simulink model "LC_DAB"  (R2025a)
settings: Solver=VariableStepAuto  StartTime=0.0  StopTime=1  RelTol=1e-3
libraries: spsVoltageMeasurementLib x5, spsCurrentMeasurementLib x4, spsIGBTDiodeLib x4, spsMosfetLib x4, spsSeriesRLCBranchLib x4, spsMeanLib x2, spsDCVoltageSourceLib x1, spsLinearTransformerLib x1, sps_lib x1
settings Model: Creator=hp  LastModifiedBy=photortist

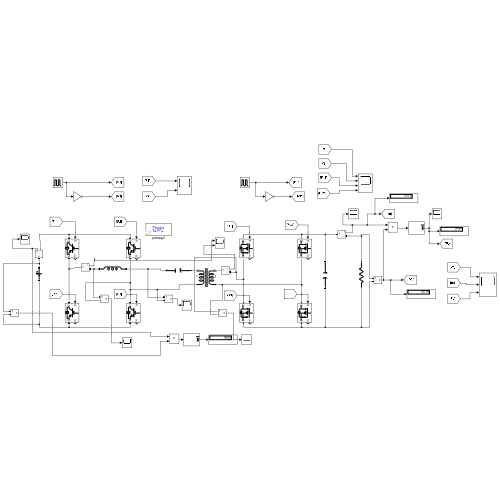
[thumbnail: Simulink's stored preview of the top-level diagram]
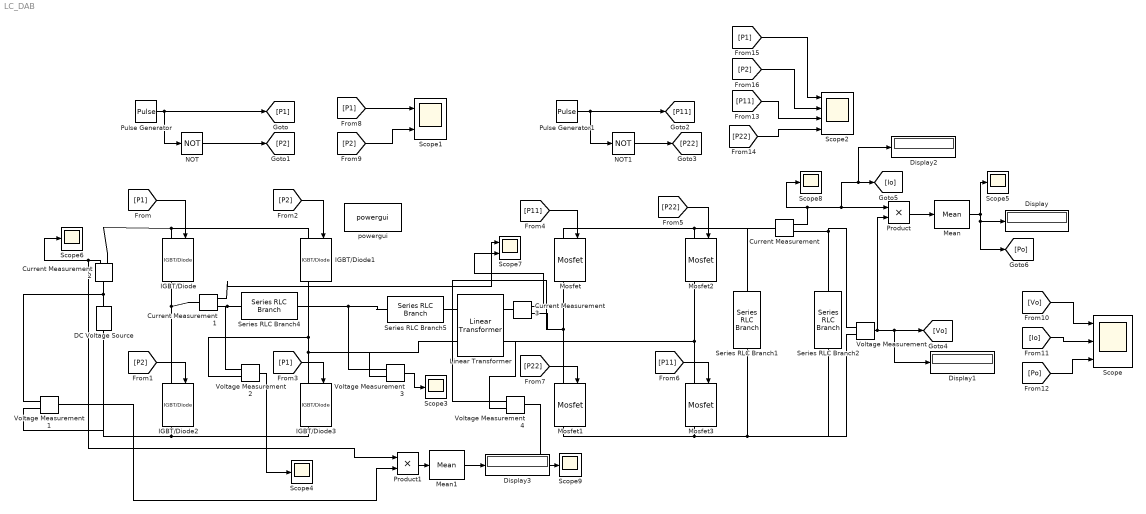
== system LC_DAB ==
  Current Measurement{,1..3} (4 alike) : spsCurrentMeasurementLib/Current Measurement  PhasorSimulation=off  OutputType=Complex  PSBequivalent=0
  DC Voltage Source : spsDCVoltageSourceLib/DC Voltage Source  Amplitude=504  Measurements=None
  Display{,1..3} (4 alike) : Display
  IGBT/Diode{,1..3} (4 alike) : spsIGBTDiodeLib/IGBT//Diode  Ron=1e-3  Rs=1e5  Cs=inf  Measurements=on
  Linear Transformer : spsLinearTransformerLib/Linear Transformer  UNITS=SI  NominalPower=[ 3000 30000 ]  winding1=[504 0 0]  winding2=[28 0 0]  ThreeWindings=off  winding3=[3.15e+05 0.7938 0.084225]  RmLm=[1.0804e+06 2866]  Measurements=None  DataType=on
  Mean : spsMeanLib/Mean  Freq=50  Vinit=0  Ts=0
  Mean1 : spsMeanLib/Mean  Freq=50  Vinit=0  Ts=0
  Mosfet{,1..3} (4 alike) : spsMosfetLib/Mosfet  Ron=0.1  Lon=0  Rd=0.01  Vfd=0  IC=0  Rs=1e5  Cs=inf  Measurements=on
  NOT : Logic  Operator=NOT  IconShape=distinctive  AllPortsSameDT=off  OutDataTypeStr=boolean
  NOT1 : Logic  Operator=NOT  IconShape=distinctive  AllPortsSameDT=off  OutDataTypeStr=boolean
  Product : Product
  Product1 : Product
  Pulse Generator : DiscretePulseGenerator  PulseType=Time based  Period=1/30000  PulseWidth=50
  Pulse Generator1 : DiscretePulseGenerator  PulseType=Time based  Period=1/30000  PulseWidth=50
  Scope : Scope  NumInputPorts=3
      settings: Title=Output Voltage  ActiveDisplayYMinimum=-3.1141163331953861  ActiveDisplayYMaximum=28.027046998758482
  Scope1 : Scope  NumInputPorts=2
      settings: ActiveDisplayYMinimum=-0.12499999999999997  ActiveDisplayYMaximum=1.125
  Scope2 : Scope  NumInputPorts=4
      settings: ActiveDisplayYMinimum=-0.12499999999999997  ActiveDisplayYMaximum=1.125  DataLoggingVariableName=ScopeData2
  Scope{3..6,8..9} (6 alike) : Scope
      Scope3 settings: ActiveDisplayYMinimum=-523.26374727748919  ActiveDisplayYMaximum=523.26375287910957  DataLoggingVariableName=ScopeData3
      Scope4 settings: ActiveDisplayYMinimum=-30.000059355602481  ActiveDisplayYMaximum=30.000032951631  DataLoggingVariableName=ScopeData4
      Scope5 settings: ActiveDisplayYMinimum=-277.72365172947951  ActiveDisplayYMaximum=2499.5128655653161  DataLoggingVariableName=ScopeData5
      Scope6 settings: ActiveDisplayYMinimum=-23.635845868791428  ActiveDisplayYMaximum=24.862575673067333  DataLoggingVariableName=ScopeData6
      Scope8 settings: ActiveDisplayYMinimum=-0.9512283756485711  ActiveDisplayYMaximum=8.5610553808371428  DataLoggingVariableName=ScopeData8
      Scope9 settings: ActiveDisplayYMinimum=-18.134641739349654  ActiveDisplayYMaximum=18.076906182134721  DataLoggingVariableName=ScopeData9
  Scope7 : Scope  NumInputPorts=2
      settings: ActiveDisplayYMinimum=-23.21316748499131  ActiveDisplayYMaximum=23.906323359507219  DataLoggingVariableName=ScopeData7
  Series RLC Branch1 : spsSeriesRLCBranchLib/Series RLC Branch  LConnTagsString=__new0  RConnTagsString=__new0  BranchType=C  Resistance=1  Inductance=1e-3  SetiL0=off  InitialCurrent=0  Capacitance=1000e-6  Setx0=off  InitialVoltage=0  Measurements=None
  Series RLC Branch2 : spsSeriesRLCBranchLib/Series RLC Branch  LConnTagsString=__new0  RConnTagsString=__new0  BranchType=R  Resistance=0.2  Inductance=1e-3  SetiL0=off  InitialCurrent=0  Capacitance=1e-6  Setx0=off  InitialVoltage=0  Measurements=None
  Series RLC Branch4 : spsSeriesRLCBranchLib/Series RLC Branch  LConnTagsString=__new0  RConnTagsString=__new0  BranchType=L  Resistance=0.01  Inductance=40e-6  SetiL0=off  InitialCurrent=0  Capacitance=1e-6  Setx0=off  InitialVoltage=0  Measurements=None
  Series RLC Branch5 : spsSeriesRLCBranchLib/Series RLC Branch  LConnTagsString=__new0  RConnTagsString=__new0  BranchType=C  Resistance=0.01  Inductance=350e-6  SetiL0=off  InitialCurrent=0  Capacitance=0.704e-6  Setx0=off  InitialVoltage=0  Measurements=None
  Voltage Measurement{,1..4} (5 alike) : spsVoltageMeasurementLib/Voltage Measurement  PhasorSimulation=off  OutputType=Complex  PSBequivalent=0
  powergui : sps_lib/powergui  Priority=1  SimulationMode=Discrete  SampleTime=0.5e-6  frequency=60  Iterations=50  frequencyindice=0  Pbase=100e6  ErrMax=1e-4  UnitsV=kV  UnitsW=MW  buscounter=0  FunctionMessages=off  echomessages=off  EnableUseOfTLC=off  CurrentSourceSwitches=off  DisableSnubberDevices=off  DisableRonSwitches=off  DisableVfSwitches=off  DisplayEquations=off  AutomaticDiscreteSolvers=off  SolverType=Tustin/Backward Euler (TBE)  Interpol=off  ExternalGateDelay=off  methode=off  Ts=100  x0status=blocks  SPID=on  SwTol=0  HookPort=off  NonlinearTolerance=1e-4  nMaxIteration=100  ContinueOnMaxIteration=off  RestoreLinks=warning  ResistiveCurrentMeasurement=off  Frange=[0:2:500]  Ylog=off  Xlog=on  ShowGrid=off  save=off  variable=ZData  structure=0  ZoomFFT=off  StartTime=0.0  cycles=1  DisplayStyle=1  fundamental=60  FreqAxis=off  MaxFrequency=1000  frequencyindicesteady=1  RmsSteady=1  display=off
  wires:
  NOT/1 -> [P2]
  [P1] -> IGBT/Diode3/1
  [P2] -> IGBT/Diode1/1
  [P1] -> IGBT/Diode/1
  [P2] -> IGBT/Diode2/1
  Voltage Measurement/1 -> Product/2, [Vo], Display1/1
  Pulse Generator/1 -> [P1], NOT/1
  Current Measurement/1 -> Scope8/1, Product/1, Display2/1, [Io]
  Product/1 -> Mean/1
  Pulse Generator1/1 -> [P11], NOT1/1
  NOT1/1 -> [P22]
  [P22] -> Mosfet1/1
  [P11] -> Mosfet3/1
  [P22] -> Mosfet2/1
  [P11] -> Mosfet/1
  [P1] -> Scope1/1
  [P2] -> Scope1/2
  [Io] -> Scope/2
  [Vo] -> Scope/1
  [Po] -> Scope/3
  [P11] -> Scope2/3
  [P22] -> Scope2/4
  Voltage Measurement3/1 -> Scope3/1
  Voltage Measurement2/1 -> Scope4/1
  Current Measurement1/1 -> Scope7/1
  Current Measurement2/1 -> Product1/1, Scope6/1
  [P2] -> Scope2/2
  [P1] -> Scope2/1
  Current Measurement3/1 -> Scope7/2
  Voltage Measurement1/1 -> Product1/2
  Product1/1 -> Mean1/1
  Mean1/1 -> Display3/1
  Mean/1 -> [Po], Display/1, Scope5/1
  Voltage Measurement4/1 -> Scope9/1
  connections:
  IGBT/Diode2/LConn1 -- Current Measurement1/LConn1 -- IGBT/Diode/RConn1
  IGBT/Diode3/LConn1 -- Voltage Measurement3/LConn2 -- Linear Transformer/LConn2 -- IGBT/Diode1/RConn1 -- Voltage Measurement2/LConn2
  IGBT/Diode/LConn1 -- Current Measurement2/RConn1 -- IGBT/Diode1/LConn1
  IGBT/Diode2/RConn1 -- DC Voltage Source/LConn1 -- Voltage Measurement1/LConn2 -- IGBT/Diode3/RConn1
  Mosfet1/LConn1 -- Voltage Measurement4/LConn1 -- Current Measurement3/RConn1 -- Mosfet/RConn1
  Mosfet/LConn1 -- Current Measurement/LConn1 -- Series RLC Branch1/LConn1 -- Mosfet2/LConn1
  Mosfet1/RConn1 -- Series RLC Branch2/RConn1 -- Voltage Measurement/LConn2 -- Series RLC Branch1/RConn1 -- Mosfet3/RConn1
  Series RLC Branch2/LConn1 -- Voltage Measurement/LConn1 -- Current Measurement/RConn1
  Voltage Measurement3/LConn1 -- Series RLC Branch5/LConn1 -- Series RLC Branch4/RConn1
  Mosfet3/LConn1 -- Voltage Measurement4/LConn2 -- Linear Transformer/RConn2 -- Mosfet2/RConn1
  DC Voltage Source/RConn1 -- Voltage Measurement1/LConn1 -- Current Measurement2/LConn1
  Linear Transformer/RConn1 -- Current Measurement3/LConn1
  Voltage Measurement2/LConn1 -- Series RLC Branch4/LConn1 -- Current Measurement1/RConn1
  Linear Transformer/LConn1 -- Series RLC Branch5/RConn1
